simulink model "easybike_battery"  (R2024a)
settings: Solver=VariableStepAuto  StartTime=0.0  StopTime=10.0  RelTol=1e-3
InitFcn:
  | if ~exist('Tbp','var'), easybike_init(1,25); end
values from neighbouring files (symbols this model uses):
  R25 = (1 - sqrt(P.RTE(c)))*P.V(c)/Iref    [easybike_discharge.m]
  Tbp = 0:5:50    [easybike_init.m]
undefined symbols (not defined in the file or in its folder): Ah_nom, CFtab, I_load, OCVtab, RFtab, SOCbp, Tcell_C
settings Model: Creator=Razowan  LastModifiedBy=Razowan

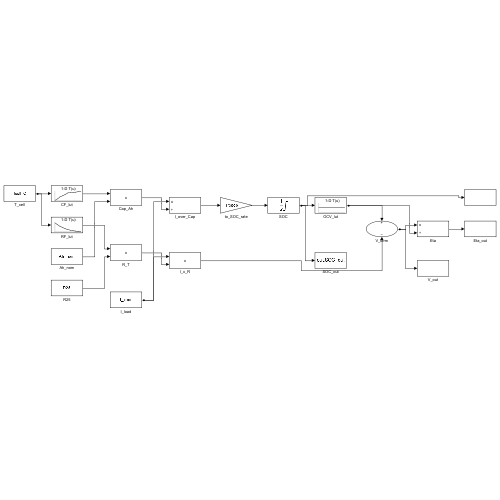
[thumbnail: Simulink's stored preview of the top-level diagram]
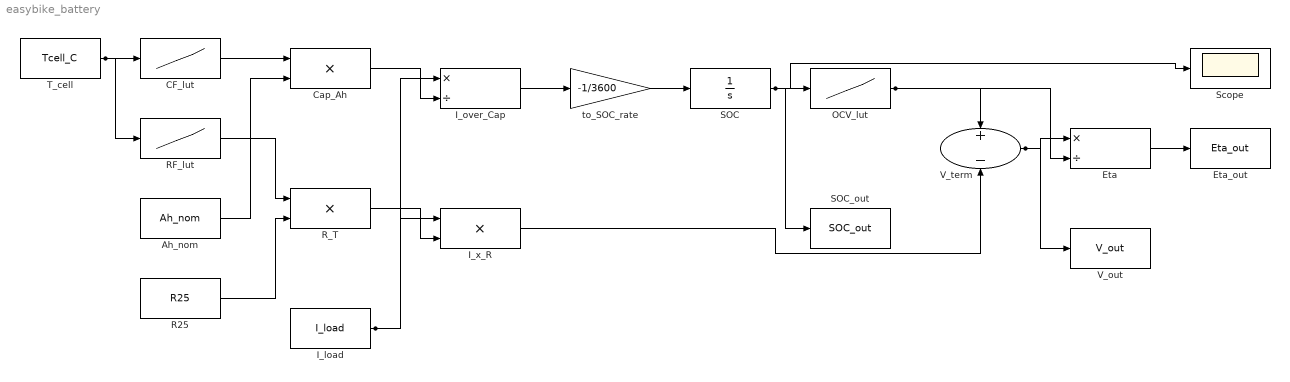
== system easybike_battery ==
  Ah_nom : Constant  Value=Ah_nom
  CF_lut : Lookup_n-D  NumberOfTableDimensions=1  BreakpointsForDimension1=Tbp  Table=CFtab  InternalRulePriority=Speed  RndMeth=Simplest
  Cap_Ah : Product  Inputs=**
  Eta : Product  Inputs=*/
  Eta_out : ToWorkspace  VariableName=Eta_out  SampleTime=-1
  I_load : Constant  Value=I_load
  I_over_Cap : Product  Inputs=*/
  I_x_R : Product  Inputs=**
  OCV_lut : Lookup_n-D  NumberOfTableDimensions=1  BreakpointsForDimension1=SOCbp  Table=OCVtab  InternalRulePriority=Speed  RndMeth=Simplest
  R25 : Constant  Value=R25
  RF_lut : Lookup_n-D  NumberOfTableDimensions=1  BreakpointsForDimension1=Tbp  Table=RFtab  InternalRulePriority=Speed  RndMeth=Simplest
  R_T : Product  Inputs=**
  SOC : Integrator  InitialCondition=1  LimitOutput=on  UpperSaturationLimit=1  LowerSaturationLimit=0
  SOC_out : ToWorkspace  VariableName=SOC_out  SampleTime=-1
  Scope : Scope
  T_cell : Constant  Value=Tcell_C
  V_out : ToWorkspace  VariableName=V_out  SampleTime=-1
  V_term : Sum  Inputs=+-
  to_SOC_rate : Gain  Gain=-1/3600
  wires:
  T_cell/1 -> CF_lut/1, RF_lut/1
  CF_lut/1 -> Cap_Ah/1
  Ah_nom/1 -> Cap_Ah/2
  RF_lut/1 -> R_T/1
  R25/1 -> R_T/2
  I_load/1 -> I_over_Cap/1, I_x_R/1
  Cap_Ah/1 -> I_over_Cap/2
  I_over_Cap/1 -> to_SOC_rate/1
  to_SOC_rate/1 -> SOC/1
  SOC/1 -> OCV_lut/1, SOC_out/1, Scope/1
  R_T/1 -> I_x_R/2
  OCV_lut/1 -> V_term/1, Eta/2
  I_x_R/1 -> V_term/2
  V_term/1 -> Eta/1, V_out/1
  Eta/1 -> Eta_out/1
